simulink model "RobotRRPlanarev2"  (R2024b)
settings: Solver=FixedStepAuto  StartTime=0.0  StopTime=100  FixedStep=0.001  RelTol=1e-3
values from neighbouring files (symbols this model uses):
  c = 340    [parameters.m]
  c1 = 0.07    [parameters.m]
  c2 = 0.1    [parameters.m]
  D = 2    [parameters.m]
  dt = 0.001    [parameters.m]
  g = 9.81    [parameters.m]
  h1 = 0.5    [parameters.m]
  h2 = 0.25    [parameters.m]
  I1 = 1/3*M1*l1^2    (= 3.33333333333)    [parameters.m]
  I2 = 1/3*M2*l2^2    (= 0.416666666667)    [parameters.m]
  l1 = 1    [parameters.m]
  l2 = 0.5    [parameters.m]
  M1 = 10    [parameters.m]
  M2 = 5    [parameters.m]
  sigma1_V = 0.1    [parameters.m]
  sigma2_V = 0.05    [parameters.m]
  sigma_W = 4    [parameters.m]
libraries: simulink x2
settings Model: Creator=Andrea  LastModifiedBy=Andrea
settings RTWCC: GPUComputeCapability=3.5

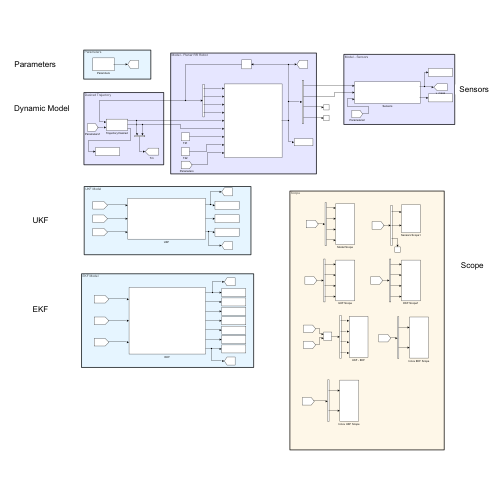
[thumbnail: Simulink's stored preview of the top-level diagram]
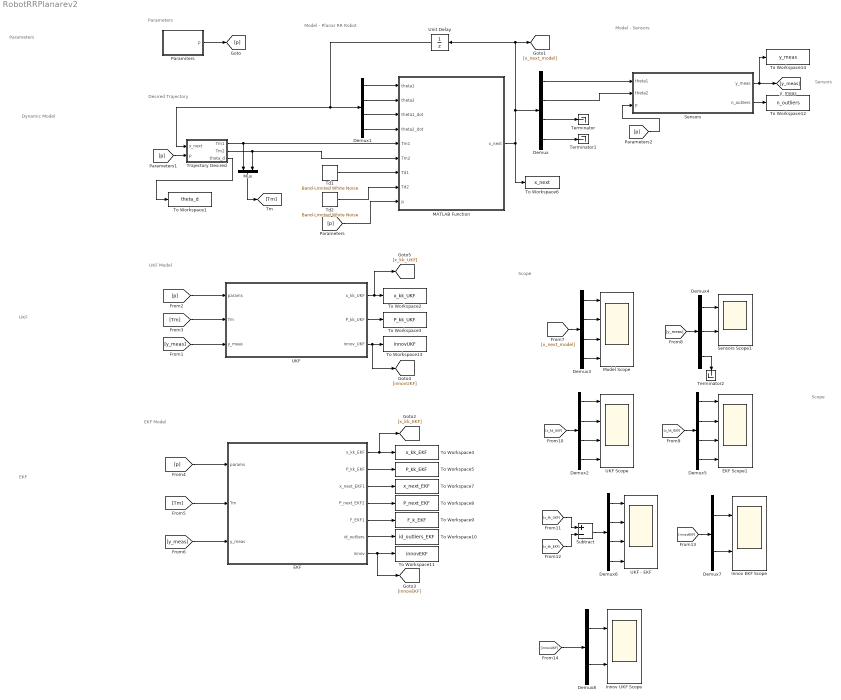
== system RobotRRPlanarev2 ==
  note: Scope
  note: Model - Sensors
  note: Model - Planar RR Robot
  note: Desired Trajectory
  note: Parameters
  note: Parameters
  note: Sensors
  note: Dynamic Model
  note: EKF Model
  note: EKF
  note: UKF Model
  note: UKF
  note: Scope
  Demux{,1..3,5..6} (6 alike) : Demux
  Demux4 : Demux  Outputs=3
  Demux7 : Demux  Outputs=2
  Demux8 : Demux  Outputs=2
  EKF : Subsystem
  EKF Scope1 : Scope  NumInputPorts=4
  Innov EKF Scope : Scope  NumInputPorts=2
  Innov UKF Scope : Scope  NumInputPorts=2
  MATLAB Function : MATLAB Function  TreatAsAtomicUnit=on  SystemSampleTime=0.001
  Model Scope : Scope  NumInputPorts=4
  Mux : Mux  Inputs=2
  Paramiters : Subsystem
  Sensors : Subsystem
  Sensors Scope1 : Scope  NumInputPorts=2
  Subtract : Sum  Inputs=+-
  Td1 : simulink/Sources/Band-Limited White Noise  Cov=[0.005]  Ts=0.001  seed=[23341]
  Td2 : simulink/Sources/Band-Limited White Noise  Cov=[0.005]  Ts=0.001  seed=[23341]
  Terminator : Terminator
  Terminator1 : Terminator
  Terminator2 : Terminator
  To Workspace1 : ToWorkspace  VariableName=theta_d  SaveFormat=Structure With Time  SampleTime=-1
  To Workspace10 : ToWorkspace  VariableName=id_outliers_EKF  SampleTime=-1
  To Workspace11 : ToWorkspace  VariableName=innovEKF  SaveFormat=Timeseries  SampleTime=-1
      settings: Save2DSignal=2-D array (concatenate along first dimension)
  To Workspace12 : ToWorkspace  VariableName=n_outliers  SampleTime=-1
  To Workspace13 : ToWorkspace  VariableName=innovUKF  SaveFormat=Timeseries  SampleTime=-1
  To Workspace14 : ToWorkspace  VariableName=y_meas  SampleTime=-1
  To Workspace2 : ToWorkspace  VariableName=x_kk_UKF  SaveFormat=Timeseries  SampleTime=-1
  To Workspace3 : ToWorkspace  VariableName=P_kk_UKF  SaveFormat=Timeseries  SampleTime=-1
  To Workspace4 : ToWorkspace  VariableName=x_kk_EKF  SaveFormat=Timeseries  SampleTime=-1
  To Workspace5 : ToWorkspace  VariableName=P_kk_EKF  SaveFormat=Timeseries  SampleTime=-1
  To Workspace6 : ToWorkspace  VariableName=x_next  SaveFormat=Timeseries  SampleTime=-1
  To Workspace7 : ToWorkspace  VariableName=x_next_EKF  SaveFormat=Timeseries  SampleTime=-1
  To Workspace8 : ToWorkspace  VariableName=P_next_EKF  SaveFormat=Timeseries  SampleTime=-1
  To Workspace9 : ToWorkspace  VariableName=F_k_EKF  SaveFormat=Timeseries  SampleTime=-1
  Trajectory Desired : Subsystem
  UKF : Subsystem
  UKF - EKF : Scope  NumInputPorts=4
  UKF Scope : Scope  NumInputPorts=4
  Unit Delay : UnitDelay  InitialCondition=[-0.7416;1.0178;0;0]  SampleTime=-1  HasFrameUpgradeWarning=on
  wires:
  Unit Delay/1 -> Trajectory Desired/1(x_next), Demux1/1
  Trajectory Desired/1(Tm1) -> Mux/1, MATLAB Function/5(Tm1)
  Trajectory Desired/2(Tm2) -> Mux/2, MATLAB Function/6(Tm2)
  Trajectory Desired/3(theta_d) -> To Workspace1/1
  [p] -> Trajectory Desired/2(p)
  Mux/1 -> [Tm]
  Td1/1 -> MATLAB Function/7(Td1)
  Td2/1 -> MATLAB Function/8(Td2)
  [p] -> MATLAB Function/9(p)
  Demux1/4 -> MATLAB Function/4(theta2_dot)
  Demux1/3 -> MATLAB Function/3(theta1_dot)
  Demux1/2 -> MATLAB Function/2(theta2)
  Demux1/1 -> MATLAB Function/1(theta1)
  Demux/1 -> Sensors/1(theta1)
  Demux/2 -> Sensors/2(theta2)
  Sensors/1(y_meas) -> To Workspace14/1, [y_meas]
  [p] -> UKF/1(params)
  [Tm] -> UKF/2(Tm)
  [y_meas] -> UKF/3(y_meas)
  UKF/1(x_kk_UKF) -> To Workspace2/1, [x_kk_UKF]
  UKF/2(P_kk_UKF) -> To Workspace3/1
  [Tm] -> EKF/2(Tm)
  [p] -> EKF/1(params)
  [y_meas] -> EKF/3(y_meas)
  EKF/2(P_kk_EKF) -> To Workspace5/1
  EKF/1(x_kk_EKF) -> To Workspace4/1, [x_kk_EKF]
  Paramiters/1(p) -> [p]
  Demux/4 -> Terminator1/1
  Demux/3 -> Terminator/1
  [x_kk_UKF] -> Demux2/1
  Demux2/1 -> UKF Scope/1
  Demux2/2 -> UKF Scope/2
  Demux2/3 -> UKF Scope/3
  Demux2/4 -> UKF Scope/4
  Demux3/4 -> Model Scope/4
  Demux3/2 -> Model Scope/2
  [x_next_model] -> Demux3/1
  Demux3/1 -> Model Scope/1
  Demux3/3 -> Model Scope/3
  Demux4/2 -> Sensors Scope1/2
  [y_meas] -> Demux4/1
  Demux4/1 -> Sensors Scope1/1
  Demux4/3 -> Terminator2/1
  Demux5/4 -> EKF Scope1/4
  Demux5/2 -> EKF Scope1/2
  [x_kk_EKF] -> Demux5/1
  Demux5/1 -> EKF Scope1/1
  Demux5/3 -> EKF Scope1/3
  MATLAB Function/1(x_next) -> [x_next_model], Unit Delay/1, Demux/1, To Workspace6/1
  [p] -> Sensors/3(p)
  [x_kk_UKF] -> Subtract/1
  [x_kk_EKF] -> Subtract/2
  Demux6/3 -> UKF - EKF/3
  Demux6/2 -> UKF - EKF/2
  Subtract/1 -> Demux6/1
  Demux6/1 -> UKF - EKF/1
  Demux6/4 -> UKF - EKF/4
  EKF/3(x_next_EKF1) -> To Workspace7/1
  EKF/4(P_next_EKF2) -> To Workspace8/1
  EKF/5(F_EKF1) -> To Workspace9/1
  EKF/6(id_outliers) -> To Workspace10/1
  Sensors/2(n_outilers) -> To Workspace12/1
  EKF/7(innov) -> [innovEKF], To Workspace11/1
  Demux7/1 -> Innov EKF Scope/1
  [innovEKF] -> Demux7/1
  Demux7/2 -> Innov EKF Scope/2
  UKF/3(innov_UKF) -> [innovUKF], To Workspace13/1
  Demux8/1 -> Innov UKF Scope/1
  [innovUKF] -> Demux8/1
  Demux8/2 -> Innov UKF Scope/2

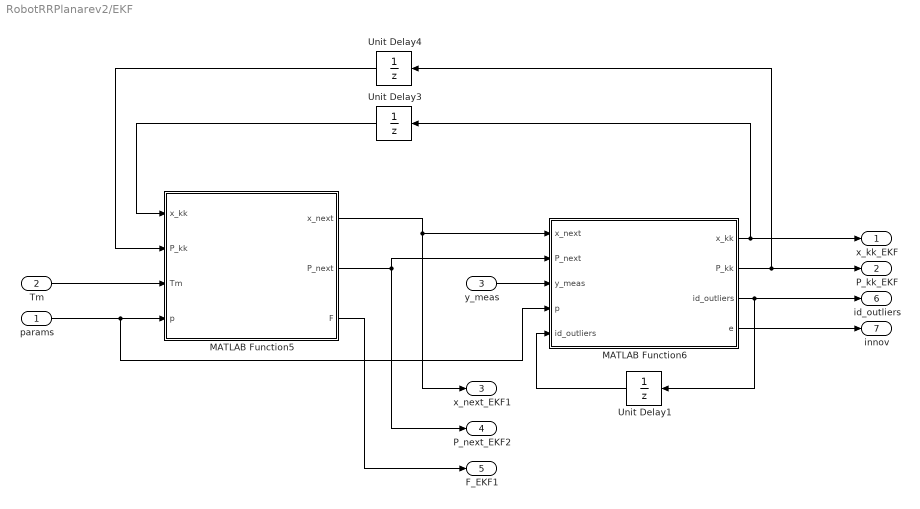
== system RobotRRPlanarev2/EKF ==
  params : Inport
  Tm : Inport  Port=2
  y_meas : Inport  Port=3
  MATLAB Function5 : MATLAB Function  TreatAsAtomicUnit=on
  MATLAB Function6 : MATLAB Function  TreatAsAtomicUnit=on
  Unit Delay1 : UnitDelay  SampleTime=-1  HasFrameUpgradeWarning=on
  Unit Delay3 : UnitDelay  InitialCondition=[-0.7416;1.0178;0;0]  SampleTime=-1  HasFrameUpgradeWarning=on
  Unit Delay4 : UnitDelay  InitialCondition=eye(4)*0  SampleTime=-1  HasFrameUpgradeWarning=on
  x_kk_EKF : Outport
  P_kk_EKF : Outport  Port=2
  x_next_EKF1 : Outport  Port=3
  P_next_EKF2 : Outport  Port=4
  F_EKF1 : Outport  Port=5
  id_outliers : Outport  Port=6
  innov : Outport  Port=7
  wires:
  Unit Delay4/1 -> MATLAB Function5/2(P_kk)
  Unit Delay3/1 -> MATLAB Function5/1(x_kk)
  MATLAB Function6/2(P_kk) -> P_kk_EKF/1, Unit Delay4/1
  MATLAB Function6/1(x_kk) -> x_kk_EKF/1, Unit Delay3/1
  params/1 -> MATLAB Function6/4(p), MATLAB Function5/4(p)
  Tm/1 -> MATLAB Function5/3(Tm)
  MATLAB Function5/1(x_next) -> x_next_EKF1/1, MATLAB Function6/1(x_next)
  MATLAB Function5/2(P_next) -> P_next_EKF2/1, MATLAB Function6/2(P_next)
  y_meas/1 -> MATLAB Function6/3(y_meas)
  MATLAB Function5/3(F) -> F_EKF1/1
  MATLAB Function6/3(id_outliers) -> Unit Delay1/1, id_outliers/1
  Unit Delay1/1 -> MATLAB Function6/5("id_outliers ")
  MATLAB Function6/4(e) -> innov/1

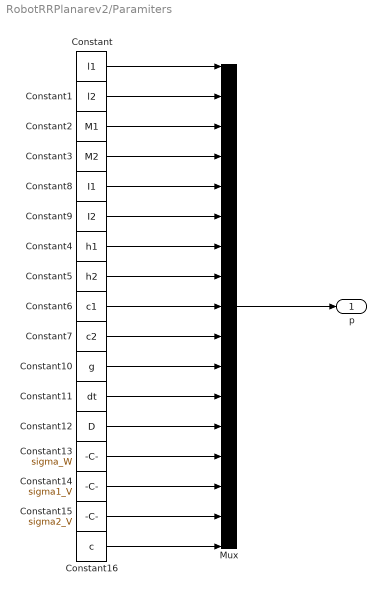
== system RobotRRPlanarev2/Paramiters ==
  Constant : Constant  Value=l1
  Constant1 : Constant  Value=l2
  Constant10 : Constant  Value=g
  Constant11 : Constant  Value=dt
  Constant12 : Constant  Value=D
  Constant13 : Constant  Value=sigma_W
  Constant14 : Constant  Value=sigma1_V
  Constant15 : Constant  Value=sigma2_V
  Constant16 : Constant  Value=c
  Constant2 : Constant  Value=M1
  Constant3 : Constant  Value=M2
  Constant4 : Constant  Value=h1
  Constant5 : Constant  Value=h2
  Constant6 : Constant  Value=c1
  Constant7 : Constant  Value=c2
  Constant8 : Constant  Value=I1
  Constant9 : Constant  Value=I2
  Mux : Mux  Inputs=17
  p : Outport
  wires:
  Mux/1 -> p/1
  Constant/1 -> Mux/1
  Constant1/1 -> Mux/2
  Constant2/1 -> Mux/3
  Constant3/1 -> Mux/4
  Constant10/1 -> Mux/11
  Constant11/1 -> Mux/12
  Constant8/1 -> Mux/5
  Constant9/1 -> Mux/6
  Constant4/1 -> Mux/7
  Constant5/1 -> Mux/8
  Constant6/1 -> Mux/9
  Constant7/1 -> Mux/10
  Constant12/1 -> Mux/13
  Constant13/1 -> Mux/14
  Constant14/1 -> Mux/15
  Constant15/1 -> Mux/16
  Constant16/1 -> Mux/17

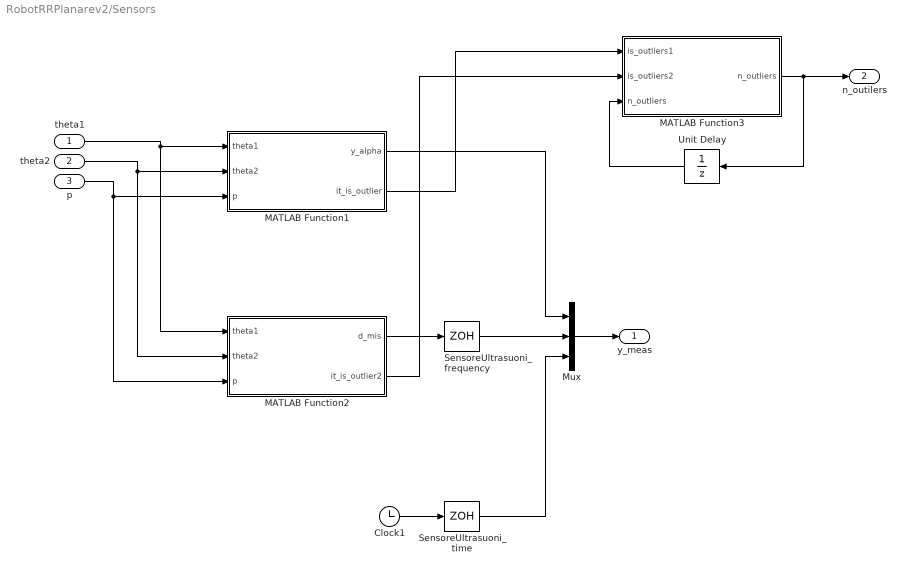
== system RobotRRPlanarev2/Sensors ==
  theta1 : Inport
  theta2 : Inport  Port=2
  p : Inport  Port=3
  Clock1 : Clock
  MATLAB Function1 : MATLAB Function  TreatAsAtomicUnit=on
  MATLAB Function2 : MATLAB Function  TreatAsAtomicUnit=on
  MATLAB Function3 : MATLAB Function  TreatAsAtomicUnit=on
  Mux : Mux  Inputs=3
  SensoreUltrasuoni_frequency : ZeroOrderHold  SampleTime=0.003
  SensoreUltrasuoni_time : ZeroOrderHold  SampleTime=0.003
  Unit Delay : UnitDelay  SampleTime=-1  HasFrameUpgradeWarning=on
  y_meas : Outport
  n_outilers : Outport  Port=2
  wires:
  theta1/1 -> MATLAB Function2/1(theta1), MATLAB Function1/1(theta1)
  theta2/1 -> MATLAB Function2/2(theta2), MATLAB Function1/2(theta2)
  Clock1/1 -> SensoreUltrasuoni_time/1
  SensoreUltrasuoni_frequency/1 -> Mux/2
  SensoreUltrasuoni_time/1 -> Mux/3
  MATLAB Function2/1(d_mis) -> SensoreUltrasuoni_frequency/1
  MATLAB Function1/1(y_alpha) -> Mux/1
  Mux/1 -> y_meas/1
  p/1 -> MATLAB Function2/3(p), MATLAB Function1/3(p)
  MATLAB Function2/2(it_is_outlier2) -> MATLAB Function3/2(is_outliers2)
  MATLAB Function1/2(it_is_outlier) -> MATLAB Function3/1(is_outliers1)
  MATLAB Function3/1(n_outliers) -> n_outilers/1, Unit Delay/1
  Unit Delay/1 -> MATLAB Function3/3("n_outliers ")

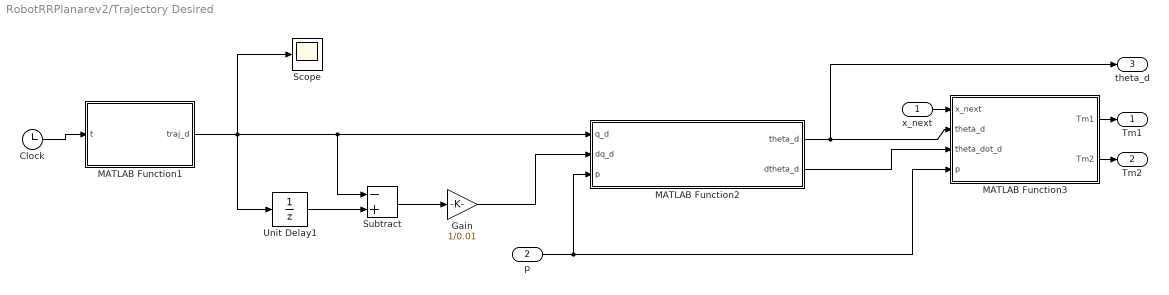
== system RobotRRPlanarev2/Trajectory Desired ==
  x_next : Inport
  p : Inport  Port=2
  Clock : Clock
  Gain : Gain  Gain=1/0.01
  MATLAB Function1 : MATLAB Function  TreatAsAtomicUnit=on
  MATLAB Function2 : MATLAB Function  TreatAsAtomicUnit=on
  MATLAB Function3 : MATLAB Function  TreatAsAtomicUnit=on
  Scope : Scope
  Subtract : Sum  Inputs=-+
  Unit Delay1 : UnitDelay  SampleTime=-1  HasFrameUpgradeWarning=on
  Tm1 : Outport
  Tm2 : Outport  Port=2
  theta_d : Outport  Port=3
  wires:
  MATLAB Function1/1(traj_d) -> Unit Delay1/1, Subtract/1, MATLAB Function2/1(q_d), Scope/1
  Unit Delay1/1 -> Subtract/2
  Subtract/1 -> Gain/1
  Clock/1 -> MATLAB Function1/1(t)
  MATLAB Function3/1(Tm1) -> Tm1/1
  Gain/1 -> MATLAB Function2/2(dq_d)
  x_next/1 -> MATLAB Function3/1(x_next)
  MATLAB Function3/2(Tm2) -> Tm2/1
  MATLAB Function2/1(theta_d) -> theta_d/1, MATLAB Function3/2(theta_d)
  MATLAB Function2/2(dtheta_d) -> MATLAB Function3/3(theta_dot_d)
  p/1 -> MATLAB Function2/3(p), MATLAB Function3/4(p)

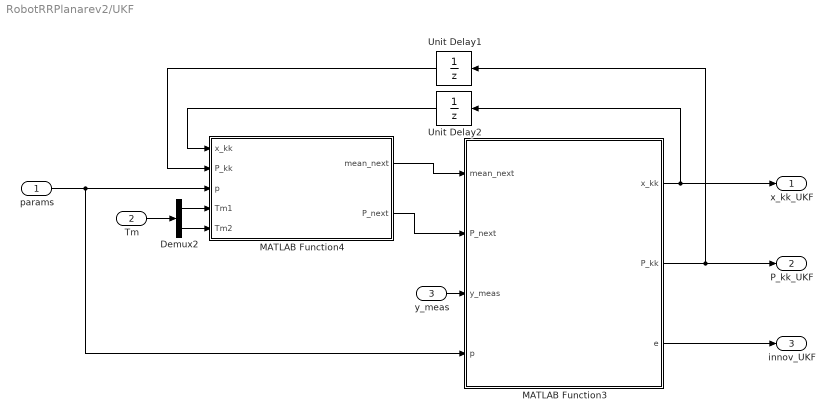
== system RobotRRPlanarev2/UKF ==
  params : Inport
  Tm : Inport  Port=2
  y_meas : Inport  Port=3
  Demux2 : Demux  Outputs=2
  MATLAB Function3 : MATLAB Function  TreatAsAtomicUnit=on
  MATLAB Function4 : MATLAB Function  TreatAsAtomicUnit=on
  Unit Delay1 : UnitDelay  InitialCondition=eye(4)*0  SampleTime=-1  HasFrameUpgradeWarning=on
  Unit Delay2 : UnitDelay  InitialCondition=[-0.7416;1.0178;0;0]  SampleTime=-1  HasFrameUpgradeWarning=on
  x_kk_UKF : Outport
  P_kk_UKF : Outport  Port=2
  innov_UKF : Outport  Port=3
  wires:
  MATLAB Function4/2(P_next) -> MATLAB Function3/2(P_next)
  MATLAB Function3/1(x_kk) -> x_kk_UKF/1, Unit Delay2/1
  Unit Delay1/1 -> MATLAB Function4/2(P_kk)
  Unit Delay2/1 -> MATLAB Function4/1(x_kk)
  Demux2/1 -> MATLAB Function4/4(Tm1)
  MATLAB Function3/2(P_kk) -> P_kk_UKF/1, Unit Delay1/1
  Demux2/2 -> MATLAB Function4/5(Tm2)
  MATLAB Function4/1(mean_next) -> MATLAB Function3/1(mean_next)
  y_meas/1 -> MATLAB Function3/3(y_meas)
  Tm/1 -> Demux2/1
  params/1 -> MATLAB Function3/4(p), MATLAB Function4/3(p)
  MATLAB Function3/3(e) -> innov_UKF/1

== matlab function RobotRRPlanarev2/EKF/MATLAB Function5 ==
  data: x_next output; P_next output; x_kk input; P_kk input; Tm input; p input; F output
function [x_next, P_next,F]  = predict_EKF(x_kk, P_kk, Tm, p)

% Definizione dei parametri del sistema
l1 = p(1)+0.2;                       % Lunghezza del link 1
l2 = p(2)+0.2;                       % Lunghezza del link 2
M1 = p(3)+0.3;                       % Massa del primo corpo
M2 = p(4)+0.2;                       % Massa del secondo corpo
I1 = p(5);                       % Momento d'inerzia del primo corpo
I2 = p(6);                       % Momento d'inerzia del secondo corpo
h1 = p(7);                       % Altezza del baricentro del primo corpo
h2 = p(8);                       % Altezza del baricentro del secondo corpo
c1 = p(9)+0.04;                       % Coefficiente di attrito viscoso per il primo link
c2 = p(10)+0.03;                      % Coefficiente di attrito viscoso per il secondo link
g = p(11);                       % Accelerazione gravitazionale (m/s^2)
dt = p(12);                      % Periodo di campionamento
sigma_W = p(14);

% Valori delle variabili dinamiche
theta1 = x_kk(1);                    % Angolo theta1
theta2 = x_kk(2);                    % Angolo theta2
theta1_dot = x_kk(3);                % Velocità angolare theta1
theta2_dot = x_kk(4);                % Velocità angolare theta2
Tm1 = Tm(1);                         % Coppia motore Tm1
Tm2 = Tm(2);                         % Coppia motore Tm2
Td1 = 0;                             % Coppia disturbo Td1
Td2 = 0;                             % Coppia disturbo Td2


F = zeros(4);

    F(1,1) = 1;
    F(2,1) = 0;
    F(3,1) = (dt*(M2*h2*l1*Td2*sin(theta1 - theta2) + M2*h2*l1*Tm2*sin(theta1 - theta2) - M2^2*h2^3*l1*theta2_dot^2*cos(theta1 - theta2) + M2^2*g*h2^2*l1*cos(theta1) + I2*M1*g*h1*cos(theta1) + I2*M2*g*l1*cos(theta1) + M2^2*h2^2*l1^2*theta1_dot^2*cos(theta1 - theta2)^2 - M2^2*h2^2*l1^2*theta1_dot^2*sin(theta1 - theta2)^2 + M1*M2*g*h1*h2^2*cos(theta1) + M2*c2*h2*l1*theta1_dot*sin(theta1 - theta2) - M2*c2*h2*l1*theta2_dot*sin(theta1 - theta2) - I2*M2*h2*l1*theta2_dot^2*cos(theta1 - theta2) + M2^2*g*h2^2*l1*sin(theta1 - theta2)*sin(theta2)))/(- M2^2*h2^2*l1^2*cos(theta1 - theta2)^2 + M2^2*h2^2*l1^2 + M1*M2*h1^2*h2^2 + I1*M2*h2^2 + I2*M2*l1^2 + I2*M1*h1^2 + I1*I2) - (2*M2^2*dt*h2^2*l1^2*cos(theta1 - theta2)*sin(theta1 - theta2)*(I2*Td1 - I2*Td2 + I2*Tm1 - I2*c1*theta1_dot - I2*c2*theta1_dot + I2*c2*theta2_dot + M2*h2^2*Td1 - M2*h2^2*Td2 + M2*h2^2*Tm1 - M2*c1*h2^2*theta1_dot - M2*c2*h2^2*theta1_dot + M2*c2*h2^2*theta2_dot - M2*h2*l1*Td2*cos(theta1 - theta2) - M2*h2*l1*Tm2*cos(theta1 - theta2) - M2^2*h2^3*l1*theta2_dot^2*sin(theta1 - theta2) + M2^2*g*h2^2*l1*sin(theta1) + I2*M1*g*h1*sin(theta1) + I2*M2*g*l1*sin(theta1) - M2*c2*h2*l1*theta1_dot*cos(theta1 - theta2) + M2*c2*h2*l1*theta2_dot*cos(theta1 - theta2) + M1*M2*g*h1*h2^2*sin(theta1) - M2^2*g*h2^2*l1*cos(theta1 - theta2)*sin(theta2) + M2^2*h2^2*l1^2*theta1_dot^2*cos(theta1 - theta2)*sin(theta1 - theta2) - I2*M2*h2*l1*theta2_dot^2*sin(theta1 - theta2)))/(- M2^2*h2^2*l1^2*cos(theta1 - theta2)^2 + M2^2*h2^2*l1^2 + M1*M2*h1^2*h2^2 + I1*M2*h2^2 + I2*M2*l1^2 + I2*M1*h1^2 + I1*I2)^2;
    F(4,1) = (dt*(M2*h2*l1*Td1*sin(theta1 - theta2) - M2*h2*l1*Td2*sin(theta1 - theta2) + M2*h2*l1*Tm1*sin(theta1 - theta2) + M2^2*h2*l1^3*theta1_dot^2*cos(theta1 - theta2) + M2^2*h2^2*l1^2*theta2_dot^2*cos(theta1 - theta2)^2 - M2^2*h2^2*l1^2*theta2_dot^2*sin(theta1 - theta2)^2 - M2*c1*h2*l1*theta1_dot*sin(theta1 - theta2) - M2*c2*h2*l1*theta1_dot*sin(theta1 - theta2) + M2*c2*h2*l1*theta2_dot*sin(theta1 - theta2) - M2^2*g*h2*l1^2*cos(theta1 - theta2)*cos(theta1) + I1*M2*h2*l1*theta1_dot^2*cos(theta1 - theta2) + M2^2*g*h2*l1^2*sin(theta1 - theta2)*sin(theta1) + M1*M2*h1^2*h2*l1*theta1_dot^2*cos(theta1 - theta2) - M1*M2*g*h1*h2*l1*cos(theta1 - theta2)*cos(theta1) + M1*M2*g*h1*h2*l1*sin(theta1 - theta2)*sin(theta1)))/(- M2^2*h2^2*l1^2*cos(theta1 - theta2)^2 + M2^2*h2^2*l1^2 + M1*M2*h1^2*h2^2 + I1*M2*h2^2 + I2*M2*l1^2 + I2*M1*h1^2 + I1*I2) - (2*M2^2*dt*h2^2*l1^2*cos(theta1 - theta2)*sin(theta1 - theta2)*(I1*Td2 + I1*Tm2 + I1*c2*theta1_dot - I1*c2*theta2_dot + M1*h1^2*Td2 + M1*h1^2*Tm2 + M2*l1^2*Td2 + M2*l1^2*Tm2 + M1*c2*h1^2*theta1_dot - M1*c2*h1^2*theta2_dot + M2*c2*l1^2*theta1_dot - M2*c2*l1^2*theta2_dot - M2*h2*l1*Td1*cos(theta1 - theta2) + M2*h2*l1*Td2*cos(theta1 - theta2) - M2*h2*l1*Tm1*cos(theta1 - theta2) + M2^2*h2*l1^3*theta1_dot^2*sin(theta1 - theta2) + M2^2*g*h2*l1^2*sin(theta2) + I1*M2*g*h2*sin(theta2) + M2*c1*h2*l1*theta1_dot*cos(theta1 - theta2) + M2*c2*h2*l1*theta1_dot*cos(theta1 - theta2) - M2*c2*h2*l1*theta2_dot*cos(theta1 - theta2) + M1*M2*g*h1^2*h2*sin(theta2) - M2^2*g*h2*l1^2*cos(theta1 - theta2)*sin(theta1) + M2^2*h2^2*l1^2*theta2_dot^2*cos(theta1 - theta2)*sin(theta1 - theta2) + I1*M2*h2*l1*theta1_dot^2*sin(theta1 - theta2) + M1*M2*h1^2*h2*l1*theta1_dot^2*sin(theta1 - theta2) - M1*M2*g*h1*h2*l1*cos(theta1 - theta2)*sin(theta1)))/(- M2^2*h2^2*l1^2*cos(theta1 - theta2)^2 + M2^2*h2^2*l1^2 + M1*M2*h1^2*h2^2 + I1*M2*h2^2 + I2*M2*l1^2 + I2*M1*h1^2 + I1*I2)^2;
    
    F(1,2) = 0;
    F(2,2) = 1;
    F(3,2) = (2*M2^2*dt*h2^2*l1^2*cos(theta1 - theta2)*sin(theta1 - theta2)*(I2*Td1 - I2*Td2 + I2*Tm1 - I2*c1*theta1_dot - I2*c2*theta1_dot + I2*c2*theta2_dot + M2*h2^2*Td1 - M2*h2^2*Td2 + M2*h2^2*Tm1 - M2*c1*h2^2*theta1_dot - M2*c2*h2^2*theta1_dot + M2*c2*h2^2*theta2_dot - M2*h2*l1*Td2*cos(theta1 - theta2) - M2*h2*l1*Tm2*cos(theta1 - theta2) - M2^2*h2^3*l1*theta2_dot^2*sin(theta1 - theta2) + M2^2*g*h2^2*l1*sin(theta1) + I2*M1*g*h1*sin(theta1) + I2*M2*g*l1*sin(theta1) - M2*c2*h2*l1*theta1_dot*cos(theta1 - theta2) + M2*c2*h2*l1*theta2_dot*cos(theta1 - theta2) + M1*M2*g*h1*h2^2*sin(theta1) - M2^2*g*h2^2*l1*cos(theta1 - theta2)*sin(theta2) + M2^2*h2^2*l1^2*theta1_dot^2*cos(theta1 - theta2)*sin(theta1 - theta2) - I2*M2*h2*l1*theta2_dot^2*sin(theta1 - theta2)))/(- M2^2*h2^2*l1^2*cos(theta1 - theta2)^2 + M2^2*h2^2*l1^2 + M1*M2*h1^2*h2^2 + I1*M2*h2^2 + I2*M2*l1^2 + I2*M1*h1^2 + I1*I2)^2 - (dt*(M2*h2*l1*Td2*sin(theta1 - theta2) + M2*h2*l1*Tm2*sin(theta1 - theta2) - M2^2*h2^3*l1*theta2_dot^2*cos(theta1 - theta2) + M2^2*h2^2*l1^2*theta1_dot^2*cos(theta1 - theta2)^2 - M2^2*h2^2*l1^2*theta1_dot^2*sin(theta1 - theta2)^2 + M2*c2*h2*l1*theta1_dot*sin(theta1 - theta2) - M2*c2*h2*l1*theta2_dot*sin(theta1 - theta2) + M2^2*g*h2^2*l1*cos(theta1 - theta2)*cos(theta2) - I2*M2*h2*l1*theta2_dot^2*cos(theta1 - theta2) + M2^2*g*h2^2*l1*sin(theta1 - theta2)*sin(theta2)))/(- M2^2*h2^2*l1^2*cos(theta1 - theta2)^2 + M2^2*h2^2*l1^2 + M1*M2*h1^2*h2^2 + I1*M2*h2^2 + I2*M2*l1^2 + I2*M1*h1^2 + I1*I2);
    F(4,2) = (2*M2^2*dt*h2^2*l1^2*cos(theta1 - theta2)*sin(theta1 - theta2)*(I1*Td2 + I1*Tm2 + I1*c2*theta1_dot - I1*c2*theta2_dot + M1*h1^2*Td2 + M1*h1^2*Tm2 + M2*l1^2*Td2 + M2*l1^2*Tm2 + M1*c2*h1^2*theta1_dot - M1*c2*h1^2*theta2_dot + M2*c2*l1^2*theta1_dot - M2*c2*l1^2*theta2_dot - M2*h2*l1*Td1*cos(theta1 - theta2) + M2*h2*l1*Td2*cos(theta1 - theta2) - M2*h2*l1*Tm1*cos(theta1 - theta2) + M2^2*h2*l1^3*theta1_dot^2*sin(theta1 - theta2) + M2^2*g*h2*l1^2*sin(theta2) + I1*M2*g*h2*sin(theta2) + M2*c1*h2*l1*theta1_dot*cos(theta1 - theta2) + M2*c2*h2*l1*theta1_dot*cos(theta1 - theta2) - M2*c2*h2*l1*theta2_dot*cos(theta1 - theta2) + M1*M2*g*h1^2*h2*sin(theta2) - M2^2*g*h2*l1^2*cos(theta1 - theta2)*sin(theta1) + M2^2*h2^2*l1^2*theta2_dot^2*cos(theta1 - theta2)*sin(theta1 - theta2) + I1*M2*h2*l1*theta1_dot^2*sin(theta1 - theta2) + M1*M2*h1^2*h2*l1*theta1_dot^2*sin(theta1 - theta2) - M1*M2*g*h1*h2*l1*cos(theta1 - theta2)*sin(theta1)))/(- M2^2*h2^2*l1^2*cos(theta1 - theta2)^2 + M2^2*h2^2*l1^2 + M1*M2*h1^2*h2^2 + I1*M2*h2^2 + I2*M2*l1^2 + I2*M1*h1^2 + I1*I2)^2 - (dt*(M2*h2*l1*Td1*sin(theta1 - theta2) - M2*h2*l1*Td2*sin(theta1 - theta2) + M2*h2*l1*Tm1*sin(theta1 - theta2) + M2^2*h2*l1^3*theta1_dot^2*cos(theta1 - theta2) - M2^2*g*h2*l1^2*cos(theta2) - I1*M2*g*h2*cos(theta2) + M2^2*h2^2*l1^2*theta2_dot^2*cos(theta1 - theta2)^2 - M2^2*h2^2*l1^2*theta2_dot^2*sin(theta1 - theta2)^2 - M1*M2*g*h1^2*h2*cos(theta2) - M2*c1*h2*l1*theta1_dot*sin(theta1 - theta2) - M2*c2*h2*l1*theta1_dot*sin(theta1 - theta2) + M2*c2*h2*l1*theta2_dot*sin(theta1 - theta2) + I1*M2*h2*l1*theta1_dot^2*cos(theta1 - theta2) + M2^2*g*h2*l1^2*sin(theta1 - theta2)*sin(theta1) + M1*M2*h1^2*h2*l1*theta1_dot^2*cos(theta1 - theta2) + M1*M2*g*h1*h2*l1*sin(theta1 - theta2)*sin(theta1)))/(- M2^2*h2^2*l1^2*cos(theta1 - theta2)^2 + M2^2*h2^2*l1^2 + M1*M2*h1^2*h2^2 + I1*M2*h2^2 + I2*M2*l1^2 + I2*M1*h1^2 + I1*I2);
        
    F(1,3) = dt;
    F(2,3) = 0; 
    F(3,3) = 1 - (dt*(I2*c1 + I2*c2 + M2*c1*h2^2 + M2*c2*h2^2 + M2*c2*h2*l1*cos(theta1 - theta2) - 2*M2^2*h2^2*l1^2*theta1_dot*cos(theta1 - theta2)*sin(theta1 - theta2)))/(- M2^2*h2^2*l1^2*cos(theta1 - theta2)^2 + M2^2*h2^2*l1^2 + M1*M2*h1^2*h2^2 + I1*M2*h2^2 + I2*M2*l1^2 + I2*M1*h1^2 + I1*I2);
    F(4,3) = (dt*(I1*c2 + M1*c2*h1^2 + M2*c2*l1^2 + 2*M2^2*h2*l1^3*theta1_dot*sin(theta1 - theta2) + M2*c1*h2*l1*cos(theta1 - theta2) + M2*c2*h2*l1*cos(theta1 - theta2) + 2*I1*M2*h2*l1*theta1_dot*sin(theta1 - theta2) + 2*M1*M2*h1^2*h2*l1*theta1_dot*sin(theta1 - theta2)))/(- M2^2*h2^2*l1^2*cos(theta1 - theta2)^2 + M2^2*h2^2*l1^2 + M1*M2*h1^2*h2^2 + I1*M2*h2^2 + I2*M2*l1^2 + I2*M1*h1^2 + I1*I2);
    
    F(1,4) = 0;
    F(2,4) = dt;
    F(3,4) = (dt*(I2*c2 + M2*c2*h2^2 - 2*M2^2*h2^3*l1*theta2_dot*sin(theta1 - theta2) + M2*c2*h2*l1*cos(theta1 - theta2) - 2*I2*M2*h2*l1*theta2_dot*sin(theta1 - theta2)))/(- M2^2*h2^2*l1^2*cos(theta1 - theta2)^2 + M2^2*h2^2*l1^2 + M1*M2*h1^2*h2^2 + I1*M2*h2^2 + I2*M2*l1^2 + I2*M1*h1^2 + I1*I2);
    F(4,4) = 1 - (dt*(- 2*theta2_dot*cos(theta1 - theta2)*sin(theta1 - theta2)*M2^2*h2^2*l1^2 + c2*cos(theta1 - theta2)*M2*h2*l1 + c2*M2*l1^2 + M1*c2*h1^2 + I1*c2))/(- M2^2*h2^2*l1^2*cos(theta1 - theta2)^2 + M2^2*h2^2*l1^2 + M1*M2*h1^2*h2^2 + I1*M2*h2^2 + I2*M2*l1^2 + I2*M1*h1^2 + I1*I2);
    
   
    %% COVARIANCE PREDICTION
   
 D = zeros(4,2);
    
    D(1,1) = 0;
    D(2,1) = 0;
    D(3,1) = (dt*(M2*h2^2 + I2))/(- M2^2*h2^2*l1^2*cos(theta1 - theta2)^2 + M2^2*h2^2*l1^2 + M1*M2*h1^2*h2^2 + I1*M2*h2^2 + I2*M2*l1^2 + I2*M1*h1^2 + I1*I2);
    D(4,1) = -(M2*dt*h2*l1*cos(theta1 - theta2))/(- M2^2*h2^2*l1^2*cos(theta1 - theta2)^2 + M2^2*h2^2*l1^2 + M1*M2*h1^2*h2^2 + I1*M2*h2^2 + I2*M2*l1^2 + I2*M1*h1^2 + I1*I2);
    
    D(1,2) = 0;
    D(2,2) = 0;
    D(3,2) = -(dt*(M2*h2^2 + M2*l1*cos(theta1 - theta2)*h2 + I2))/(- M2^2*h2^2*l1^2*cos(theta1 - theta2)^2 + M2^2*h2^2*l1^2 + M1*M2*h1^2*h2^2 + I1*M2*h2^2 + I2*M2*l1^2 + I2*M1*h1^2 + I1*I2);
    D(4,2) = (dt*(M1*h1^2 + M2*l1^2 + M2*h2*cos(theta1 - theta2)*l1 + I1))/(- M2^2*h2^2*l1^2*cos(theta1 - theta2)^2 + M2^2*h2^2*l1^2 + M1*M2*h1^2*h2^2 + I1*M2*h2^2 + I2*M2*l1^2 + I2*M1*h1^2 + I1*I2);


% Stima Predizione
% Matrice di massa
M = [I1 + M1*h1^2 + M2*l1^2, l1*M2*h2*cos(theta1 - theta2);
     l1*M2*h2*cos(theta1 - theta2), I2 + M2*h2^2];

% Matrice N
N = [c1 + c2, -c2;
     -c2, c2];

% Vettore q
q = [l1*M2*h2*sin(theta1 - theta2)*theta2_dot^2 - (M1*h1 + M2*l1)*g*sin(theta1);
     -l1*M2*h2*sin(theta1 - theta2)*theta1_dot^2 - M2*h2*g*sin(theta2)];

% Matrice G
G = [1, 0;
     0, 1];

% Matrice T
T = [1, -1;
     0,  1];

% Calcolo accelerazioni
theta_ddot = pinv(M) * (G * [Tm1; Tm2] + T * [Td1; Td2] - N * [theta1_dot; theta2_dot] - q);

x_next = zeros(4,1);

% Aggiornamento degli stati con Eulero
x_next(1) = theta1 + theta1_dot * dt;
x_next(2) = theta2 + theta2_dot * dt;
x_next(3) = theta1_dot + theta_ddot(1) * dt;
x_next(4) = theta2_dot + theta_ddot(2) * dt;

% Covarianza Errore Predizione
Q = [sigma_W^2, 0; 0, sigma_W^2]; 
Q = T * Q * T';
% Qp = eye(4) * 0.001;
P_next = F * P_kk * F' + D * Q * D';

end

== matlab function RobotRRPlanarev2/EKF/MATLAB Function6 ==
  data: x_kk output; P_kk output; x_next input; P_next input; y_meas input; p input; id_outliers input; id_outliers output; e output
function [x_kk, P_kk, id_outliers, e]  = correct_EKF(x_next, P_next, y_meas, p, id_outliers)

    MAHALANOBIS = true;
    mahalanobis_threshold = 4;
    
    % Definizione dei parametri del sistema
    l1 = p(1);                       % Lunghezza del link 1
    l2 = p(2);                       % Lunghezza del link 2
    M1 = p(3);                       % Massa del primo corpo
    M2 = p(4);                       % Massa del secondo corpo
    I1 = p(5);                       % Momento d'inerzia del primo corpo
    I2 = p(6);                       % Momento d'inerzia del secondo corpo
    h1 = p(7);                       % Altezza del baricentro del primo corpo
    h2 = p(8);                       % Altezza del baricentro del secondo corpo
    c1 = p(9);                       % Coefficiente di attrito viscoso per il primo link
    c2 = p(10);                      % Coefficiente di attrito viscoso per il secondo link
    g = p(11);                       % Accelerazione gravitazionale (m/s^2)
    dt = p(12);                      % Periodo di campionamento
    D = p(13);
    sigma1_V = p(15);
    sigma2_V = p(16);

    R = [sigma1_V^2, 0; 0, sigma2_V^2];
    
    % Valori delle variabili dinamiche
    theta1 = x_next(1);                    % Angolo theta1
    theta2 = x_next(2);                    % Angolo theta2
    theta1_dot = x_next(3);                 % Velocità angolare theta1
    theta2_dot = x_next(4);                 % Velocità angolare theta2
    v1 = 0;
    v2 = 0;
    
    if (x_next(1) > 0)
        H = [-1, 1, 0, 0;
             -l1*cos(theta1), 0, 0, 0
            ];
    
        Mh = eye(2);
    else
        H = [1, -1, 0, 0;
             l1*cos(theta1), 0, 0, 0
             ];
    
        Mh = eye(2);
    end
    
    
    T_sens = y_meas(3);
    y_meas = y_meas(1:2);
    
    y_cor = zeros(2,1);
    
    if (x_next(1) > 0)
        ang_mis = pi - x_next(1) + x_next(2);
        x = D - l1 * sin(x_next(1));
    else
        ang_mis = pi + x_next(1) - x_next(2);
        x = D + l1 * sin(x_next(1));
    end  
    y_cor(1) = ang_mis + v1;
    y_cor(2) = x + v2;

    e = y_meas - y_cor;
    e(1,1) = atan2(sin(e(1,1)),cos(e(1,1)));
    S_k = H * P_next * H' + Mh * R * Mh';
    L_k = P_next * H' / (S_k);
    mahalanobis_distance = sqrt(e' / (S_k) * e);
            
    if mahalanobis_distance>mahalanobis_threshold && MAHALANOBIS
          x_kk = x_next;
          P_kk = P_next;
          id_outliers = id_outliers + 1;
    else
          x_kk = x_next + L_k * (e);
          P_kk = (eye(4) - L_k * H) * P_next * (eye(4) - L_k * H)' + L_k * Mh * (R) * Mh' * L_k';    % Joseph formula for Covariance Correction
    end
end

== matlab function RobotRRPlanarev2/Sensors/MATLAB Function3 ==
  data: is_outliers1 input; is_outliers2 input; n_outliers output; n_outliers input
function n_outliers  = outliers(is_outliers1, is_outliers2, n_outliers)

    if (is_outliers1) || is_outliers2
        n_outliers = n_outliers + 1;
    end
end

== matlab function RobotRRPlanarev2/Trajectory Desired/MATLAB Function1 ==
  data: t input; traj_d output
function traj_d = trajectory(t)
    % Parametri della traiettoria
    a = 0.25;         % Semi-asse maggiore (raggio lungo l'asse X)
    b = 0.25;        % Semi-asse minore (raggio lungo l'asse Y)
        
    X_c = 0;      % Centro X
    Y_c = 1;      % Centro Y
    omega = - 0.5;   % Velocità angolare

    % Posizione X e Y desiderata
    X_d = X_c + a * cos(omega * t);   % Posizione X
    Y_d = Y_c + b * sin(omega * t);   % Posizione Y

    % Posizione desiderata (output)
    traj_d = [X_d; Y_d];
    
end

== matlab function RobotRRPlanarev2/MATLAB Function ==
  data: theta1 input; theta2 input; x_next output; theta1_dot input; theta2_dot input; Tm1 input; Tm2 input; Td1 input; Td2 input; p input
function x_next = model_discrete(theta1, theta2, theta1_dot, theta2_dot, Tm1, Tm2, Td1, Td2, p)

    % Definizione dei parametri del sistema
    l1 = p(1);                       % Lunghezza del link 1
    l2 = p(2);                       % Lunghezza del link 2
    M1 = p(3);                       % Massa del primo corpo
    M2 = p(4);                       % Massa del secondo corpo
    I1 = p(5);                       % Momento d'inerzia del primo corpo
    I2 = p(6);                       % Momento d'inerzia del secondo corpo
    h1 = p(7);                       % Altezza del baricentro del primo corpo
    h2 = p(8);                       % Altezza del baricentro del secondo corpo
    c1 = p(9);                       % Coefficiente di attrito viscoso per il primo link
    c2 = p(10);                      % Coefficiente di attrito viscoso per il secondo link
    g = p(11);                       % Accelerazione gravitazionale (m/s^2)
    dt = p(12);                      % Periodo di campionamento

    % Matrice di massa M(ϑ)
    M = [I1 + M1 * h1^2 + M2 * l1^2, l1 * M2 * h2 * cos(theta1 - theta2);
         l1 * M2 * h2 * cos(theta1 - theta2), I2 + M2 * h2^2];
    
    % Matrice N
    N = [c1 + c2, -c2;
         -c2, c2];
    
    % Vettore q(ϑ)
    q = [l1 * M2 * h2 * sin(theta1 - theta2) * theta2_dot^2 - (M1 * h1 + M2 * l1) * g * sin(theta1);
         -l1 * M2 * h2 * sin(theta1 - theta2) * theta1_dot^2 - M2 * h2 * g * sin(theta2)];
    
    % Matrice G
    G = [1, 0;
         0, 1];
    
    % Matrice T
    T = [1, -1;
         0,  1];
    
    % Calcolo accelerazioni
    theta_ddot = pinv(M) * (G * [Tm1; Tm2] + T * [Td1; Td2] - N * [theta1_dot; theta2_dot] - q);
    
    % Aggiornamento degli stati con Eulero
    theta1_next = theta1 + theta1_dot * dt;
    theta2_next = theta2 + theta2_dot * dt;
    theta1_dot_next = theta1_dot + theta_ddot(1) * dt;
    theta2_dot_next = theta2_dot + theta_ddot(2) * dt;
    
    % Stato successivo
    x_next = [theta1_next;
              theta2_next;
              theta1_dot_next;
              theta2_dot_next];
end

== matlab function RobotRRPlanarev2/Trajectory Desired/MATLAB Function2 ==
  data: q_d input; theta_d output; dtheta_d output; dq_d input; p input
function [theta_d, dtheta_d] = inverse_kinematics(q_d, dq_d,p)

     % Definizione dei parametri del sistema
    l1 = p(1);                       % Lunghezza del link 1
    l2 = p(2);                       % Lunghezza del link 2
    M1 = p(3);                       % Massa del primo corpo
    M2 = p(4);                       % Massa del secondo corpo
    I1 = p(5);                       % Momento d'inerzia del primo corpo
    I2 = p(6);                       % Momento d'inerzia del secondo corpo
    h1 = p(7);                       % Altezza del baricentro del primo corpo
    h2 = p(8);                       % Altezza del baricentro del secondo corpo
    c1 = p(9);                       % Coefficiente di attrito viscoso per il primo link
    c2 = p(10);                      % Coefficiente di attrito viscoso per il secondo link
    g = p(11);                       % Accelerazione gravitazionale (m/s^2)
    dt = p(12);                      % Periodo di campionamento
        
    x = q_d(1);  % x-coordinate of the desired position
    y = q_d(2);  % y-coordinate of the desired position
    
    % Check for reachability (if the position is within the robot's workspace)
    if sqrt(x^2 + y^2) > (l1 + l2)
        error('Position not reachable: exceeds range of arm');
    end
    
    % Compute theta2 (relative angle of the second joint)
    % cos_theta2 = (x^2 + y^2 - l1^2 - l2^2) / (2 * l1 * l2);
    % sin_theta2 = sqrt(1 - cos_theta2^2);  % Positive by convention (elbow-up solution)
    % theta2 = atan2(sin_theta2, cos_theta2);
    
    % Compute theta1 (absolute angle of the first joint)
    % phi = atan2(x, y);  % Angle towards the desired point
    % beta = atan2(l2 * sin_theta2, l1 + l2 * cos_theta2);  % Compensation angle
    % theta1 = phi - beta;

    theta1 = 2*atan(((l2^2*(2*l2*x - ((- l1^2 + 2*l1*l2 - l2^2 + x^2 + y^2)*(l1^2 + 2*l1*l2 + l2^2 - x^2 - y^2))^(1/2)))/(- l1^2 + l2^2 + 2*l2*y + x^2 + y^2) - 2*l2*x - (l1^2*(2*l2*x - ((- l1^2 + 2*l1*l2 - l2^2 + x^2 + y^2)*(l1^2 + 2*l1*l2 + l2^2 - x^2 - y^2))^(1/2)))/(- l1^2 + l2^2 + 2*l2*y + x^2 + y^2) - 2*l1*x + (x^2*(2*l2*x - ((- l1^2 + 2*l1*l2 - l2^2 + x^2 + y^2)*(l1^2 + 2*l1*l2 + l2^2 - x^2 - y^2))^(1/2)))/(- l1^2 + l2^2 + 2*l2*y + x^2 + y^2) + (y^2*(2*l2*x - ((- l1^2 + 2*l1*l2 - l2^2 + x^2 + y^2)*(l1^2 + 2*l1*l2 + l2^2 - x^2 - y^2))^(1/2)))/(- l1^2 + l2^2 + 2*l2*y + x^2 + y^2) + (2*l2*y*(2*l2*x - ((- l1^2 + 2*l1*l2 - l2^2 + x^2 + y^2)*(l1^2 + 2*l1*l2 + l2^2 - x^2 - y^2))^(1/2)))/(- l1^2 + l2^2 + 2*l2*y + x^2 + y^2))/(l1^2 + 2*l1*y - l2^2 + x^2 + y^2));

    theta2 = -2*atan((2*l2*x - ((- l1^2 + 2*l1*l2 - l2^2 + x^2 + y^2)*(l1^2 + 2*l1*l2 + l2^2 - x^2 - y^2))^(1/2))/(- l1^2 + l2^2 + 2*l2*y + x^2 + y^2));

    
    % Result: joint angles
    theta_d = [theta1; theta2]; 
    
    % Jacobian matrix 
    J = [-l1 * cos(theta1), -l2 * cos(theta2);...
         -l1 * sin(theta1), -l2 * sin(theta2)];
    
    % Inverse Jacobian 
    J_inv = pinv(J);
    
    % Compute the joint velocities (dtheta_d) using the inverse Jacobian
    dtheta_d = J_inv * dq_d;

end

== matlab function RobotRRPlanarev2/Trajectory Desired/MATLAB Function3 ==
  data: x_next input; Tm1 output; theta_d input; theta_dot_d input; Tm2 output; p input
function [Tm1, Tm2] = pd_control(x_next, theta_d, theta_dot_d, p)

     % Definizione dei parametri del sistema
    l1 = p(1);                       % Lunghezza del link 1
    l2 = p(2);                       % Lunghezza del link 2
    M1 = p(3);                       % Massa del primo corpo
    M2 = p(4);                       % Massa del secondo corpo
    I1 = p(5);                       % Momento d'inerzia del primo corpo
    I2 = p(6);                       % Momento d'inerzia del secondo corpo
    h1 = p(7);                       % Altezza del baricentro del primo corpo
    h2 = p(8);                       % Altezza del baricentro del secondo corpo
    c1 = p(9);                       % Coefficiente di attrito viscoso per il primo link
    c2 = p(10);                      % Coefficiente di attrito viscoso per il secondo link
    g = p(11);                       % Accelerazione gravitazionale (m/s^2)
    dt = p(12);                      % Periodo di campionamento

    theta = x_next(1:2);
    theta_dot = x_next(3:4);

    
    % Control parameters
    kp = 20;  % Proportional gain
    kd = 10;  % Derivative gain
    
    % Calculate the errors in position and velocity
    e = theta_d - theta;     % Position error
    e_dot = theta_dot_d - theta_dot;  % Velocity error
    
    % Gravity vector calculation
    G = [- (M1 * h1 + M2 * l1) * g * sin(theta(1));...
         - (M2 * h2) * g * sin(theta(2))];
    
   % PD control input + gravity compensation
    tau = kd * e_dot + kp * e + G;

    Tm1 = tau(1);
    Tm2 = tau(2);

end

== matlab function RobotRRPlanarev2/Sensors/MATLAB Function1 ==
  data: theta1 input; y_alpha output; theta2 input; p input; it_is_outlier output
function [y_alpha, it_is_outlier] = EncoderOttico(theta1, theta2, p)

    % Parametri
    sigma_encoder = p(15);  % Deviazione std rumore encoder
    
    % Misura
    if (theta1 > 0)
        ang_mis = pi - theta1 + theta2;
    else
        ang_mis = pi + theta1 - theta2;
    end

    % Rumore di misura encoder
    v_encoder = sigma_encoder * randn;
    
    % Generazione outlier
    it_is_outlier = (rand(1,1) < 0.01); 
        
    % Modello di misura encoder
    y_alpha =  ang_mis + v_encoder + 50 * (rand(1,1) - 0.5) * it_is_outlier;  

end

== matlab function RobotRRPlanarev2/Sensors/MATLAB Function2 ==
  data: theta1 input; d_mis output; theta2 input; p input; it_is_outlier2 output
function [d_mis, it_is_outlier2] = SensoreUltrasuoni(theta1, theta2, p)

    % parametri
    l1 = 1;
    D = p(13);        %m
    c = p(17);      %[m/s]
    
    % caratterizzazione
    sensor_noise_sigma = p(16);       %[s]
    sensor_t = 0.01;                %tempo di discretizzazione [s]
    dT = sensor_t;                  %loop period is sensor period

    %misura
    if (theta1 > 0)
        x = D - l1 * sin(theta1);
    else 
        x = D + l1 * sin(theta1);
    end

    % Generazione outlier
    it_is_outlier2 = (rand(1,1) < 0.01);
    
    d_mis = x + sensor_noise_sigma.*randn + 50 * (rand(1,1) - 0.5) * it_is_outlier2;
  
end

== matlab function RobotRRPlanarev2/UKF/MATLAB Function3 ==
  data: mean_next input size=[4,1]; x_kk output size=[4,1]; P_next input size=[4,4]; P_kk output size=[4,4]; y_meas input size=[3,1]; p input; e output
function [x_kk, P_kk, e] = UKF_correction(mean_next, P_next, y_meas, p)

    MAHALANOBIS = true;
    mahalanobis_threshold = 4;
    
    D = 2;

    l1 = p(1);                       % Lunghezza del link 1
    dt = p(12);                      % Periodo di campionamento
    sigma1_V = p(15);
    sigma2_V = p(16);

    R = [sigma1_V^2, 0; 0, sigma2_V^2];       

    T_sens = y_meas(3);
    y_meas = [y_meas(1);y_meas(2)];

    % define paramenters
    alpha = 1;            % not scaled
    beta = 2;             % optimum for the Gaussian case
    kappa = 0;            % lambda = 0 [weight of the central sigma_point]
    
    enne = size(mean_next,1);
    
    lambda = alpha^2*(enne + kappa) - enne;
    
    % compute weights
    wc = zeros(1, 2 * enne + 1);
    w0 = lambda/(lambda + enne);
    wc(1) = w0 + 1 - alpha^2 + beta;      %secondo ordine
    wc(2:2*enne+1) = 1/2/(enne+lambda);
    
    wm = wc;                              %primo ordine
    wm(1) = w0;
    
    % factorise covariance matrix
    % SVD
    [U,S,~] = svd(P_next);
    GAMMA = U*sqrt(S);
    
    % generate 2n+1 sigma points
    sigma_points = zeros(enne, 2*enne+1);
    sigma_points(:,1) = mean_next;
    for i = 1:size(GAMMA,2)
        sigma_points(:,i+1)      =  mean_next + sqrt(enne+lambda)*GAMMA(:,i);
        sigma_points(:,i+1+enne) =  mean_next - sqrt(enne+lambda)*GAMMA(:,i);
    end
    
    %% apply function h to the 2n+1 sigma points
    y_cor = zeros(2,size(sigma_points,2));
    for i=1:size(sigma_points,2)
        if (sigma_points(1,i) > 0)
            ang_mis = pi - sigma_points(1,i) + sigma_points(2,i);
        else
            ang_mis = pi + sigma_points(1,i) - sigma_points(2,i);
        end 
        y_cor(1,i) =  ang_mis;
        
        if (sigma_points(1,i) > 0)
            x = D - l1 * sin(sigma_points(1,i));
        else 
            x = D + l1 * sin(sigma_points(1,i));
        end
        y_cor(2,i) = x;
        
    end

    % compute propagated mean
    ymean_next = zeros(2,1);
    ymean_next(2,1) = y_cor(2,:)*wm';
    ymean_next(1,1) = atan2(sin(y_cor(1,:))*wm',cos(y_cor(1,:))*wm');
    
    % propagated ~
    ytilde_next =  y_cor - ymean_next;
    ytilde_next(1, :) = atan2(sin(ytilde_next(1, :)), cos(ytilde_next(1, :)));
    xtilde_next = sigma_points - mean_next;
    xtilde_next(1, :) = atan2(sin(xtilde_next(1, :)), cos(xtilde_next(1, :)));

    % compute virtual measurements second order
    S_k = zeros(2,2);
    cross_cov = zeros(enne,2);
    for i = 1:size(sigma_points,2)
        S_k = S_k + wc(i)*ytilde_next(:,i)*ytilde_next(:,i)';
        cross_cov = cross_cov + wc(i) * (xtilde_next(:,i) * ytilde_next(:,i)');
    end
   
    e = y_meas - ymean_next;
    e(1,1) = atan2(sin(e(1,1)),cos(e(1,1)));
    S_k = S_k + R;
    L_k = cross_cov * pinv(S_k);
    mahalanobis_distance = sqrt(e' * pinv(S_k) * e);
        
    if mahalanobis_distance>mahalanobis_threshold && MAHALANOBIS
        x_kk = mean_next;
        P_kk = P_next;
        %number_of_identified_outliers = number_of_identified_outliers + 1;
        identified_outlier = 1;
    else
        x_kk = mean_next + L_k * (e);
        P_kk = P_next - L_k * S_k * L_k';
        %P_c = (eye(size(x_hat,1)) - L*C) * P * (eye(size(x_hat,1)) - L*C)' + L*R*L';    % Joseph formula for Covariance Correction
    end
end

== matlab function RobotRRPlanarev2/UKF/MATLAB Function4 ==
  data: x_kk input size=[4,1]; P_kk input size=[4,4]; p input size=[17,1]; Tm1 input size=1; Tm2 input size=1; mean_next output size=[4,1]; P_next output size=[4,4]
function [mean_next, P_next] = UKF_prediction(x_kk,P_kk, p, Tm1, Tm2)

    % Definizione dei parametri del sistema
    l1 = p(1);                       % Lunghezza del link 1
    l2 = p(2);                       % Lunghezza del link 2
    M1 = p(3);                       % Massa del primo corpo
    M2 = p(4);                       % Massa del secondo corpo
    I1 = p(5);                       % Momento d'inerzia del primo corpo
    I2 = p(6);                       % Momento d'inerzia del secondo corpo
    h1 = p(7);                       % Altezza del baricentro del primo corpo
    h2 = p(8);                       % Altezza del baricentro del secondo corpo
    c1 = p(9);                       % Coefficiente di attrito viscoso per il primo link
    c2 = p(10);                      % Coefficiente di attrito viscoso per il secondo link
    g = p(11);                       % Accelerazione gravitazionale (m/s^2)
    dt = p(12);                      % Periodo di campionamento
    sigma_W = p(14);

    x_kk = [x_kk;0;0];
    Q = [sigma_W^2, 0; 0, sigma_W^2]; 
    P_kk = blkdiag(P_kk, Q);
    % Qp = eye(4)*0.001;

    % define paramenters
    alpha = 1;            % not scaled
    beta = 2;             % optimum for the Gaussian case
    kappa = 0;            % lambda = 0 [weight of the central sigma_point]
    
    enne = size(x_kk,1);
    
    lambda = alpha^2*(enne + kappa) - enne;
    
    % compute weights
    wc = zeros(1, 2 * enne + 1);
    w0 = lambda/(lambda + enne);
    wc(1) = w0 + 1 - alpha^2 + beta;      %secondo ordine
    wc(2:2*enne+1) = 1/2/(enne+lambda);
    
    wm = wc;                              %primo ordine
    wm(1) = w0;
    
    % factorise covariance matrix
    % SVD
    [U,S,~] = svd(P_kk);
    GAMMA = U*sqrt(S);
    
    % generate 2n+1 sigma points
    sigma_points = zeros(enne, 2*enne+1);
    sigma_points(:,1) = x_kk;
    for i = 1:size(GAMMA,2)
        sigma_points(:,i+1)      =  x_kk + sqrt(enne+lambda)*GAMMA(:,i);
        sigma_points(:,i+1+enne) =  x_kk - sqrt(enne+lambda)*GAMMA(:,i);
    end
    
    %% apply function f to the 2n+1 sigma points
    sigma_points_next = zeros(4,size(sigma_points,2));
    for i=1:size(sigma_points,2)
        % Matrice di massa M(ϑ)
        M = [I1 + M1 * h1^2 + M2 * l1^2, l1 * M2 * h2 * cos(sigma_points(1,i) - sigma_points(2,i));
             l1 * M2 * h2 * cos(sigma_points(1,i) - sigma_points(2,i)), I2 + M2 * h2^2];
        
        % Matrice N
        N = [c1 + c2, -c2;
             -c2, c2];
        
        % Vettore q(ϑ)
        q = [l1 * M2 * h2 * sin(sigma_points(1,i) - sigma_points(2,i)) * (sigma_points(4,i))^2 - (M1 * h1 + M2 * l1) * g * sin(sigma_points(1,i));
             -l1 * M2 * h2 * sin(sigma_points(1,i) - sigma_points(2,i)) * (sigma_points(3,i))^2 - M2 * h2 * g * sin(sigma_points(2,i))];
        
        % Matrice G
        G = [1, 0;
             0, 1];
        
        % Matrice T
        T = [1, -1;
             0,  1];
      
        theta_ddot = pinv(M) * (G * [Tm1; Tm2] + T * [sigma_points(5,i); sigma_points(6,i)] - N * [sigma_points(3,i); sigma_points(4,i)] - q);
        sigma_points_next(1,i) = sigma_points(1,i) + sigma_points(3,i) * dt;
        sigma_points_next(2,i) = sigma_points(2,i) + sigma_points(4,i) * dt;
        sigma_points_next(3,i) = sigma_points(3,i) + theta_ddot(1,1) * dt;
        sigma_points_next(4,i) = sigma_points(4,i) + theta_ddot(2,1) * dt;
    end
    
    % compute propagated mean
    mean_next = zeros(4,1);
    mean_next(1,1) = atan2(sin(sigma_points_next(1,:))*wm',cos(sigma_points_next(1,:))*wm');
    mean_next(2,1) = atan2(sin(sigma_points_next(2,:))*wm',cos(sigma_points_next(2,:))*wm');
    mean_next(3,1) = sigma_points_next(3,:)*wm';
    mean_next(4,1) = sigma_points_next(4,:)*wm';

    % propagated ~
    tilde_next = sigma_points_next - mean_next;
    tilde_next(1:2, :) = atan2(sin(tilde_next(1:2, :)), cos(tilde_next(1:2, :)));

    % compute virtual measurements second order
    P_next = zeros(4,4);
    for i = 1:size(sigma_points,2)
        P_next = P_next + wc(i)*(tilde_next(:,i)*tilde_next(:,i)');
    end
    P_next = P_next;

end
